simulink model "Motor_IMU_Test"  (R2026a)
settings: Solver=FixedStepAuto  StopTime=10  FixedStep=.001  EnableMultiTasking=on
InitFcn:
  | addpath('C:\Users\jpgre\OneDrive\Documents\ChatGPT\ETE 4851 Project\outputs\motor_imu');
libraries: stm32f4xxblockslib x4, stm32blockslib x3
settings Model: STM32="{\"DigitalPortWrite\":[{\"ID\":\"92\"},{\"ID\":\"93\"},{\"ID\":\"116\"}],\"PWMOutput\":{\"ID\":\"91\"},\"UARTWrite\":[{\"ID\":\"103\"},{\"ID\":\"110\"}],\"UARTRead\":{\"ID\":\"98\"}}"  SimulationMode=external  ExtModeTrigDuration=10  Creator=smboskovich  LastModifiedBy=jpgre
settings OptimizationCC: PassReuseOutputArgsThreshold=0.0  MaxStackSize=512
settings HardwareCC: ProdLargestAtomicInteger=Long  ProdLargestAtomicFloat=Double  ProdHWDeviceType=ARM Compatible->ARM Cortex-M
settings RTWCC: SystemTargetFile=ert.tlc  HardwareBoard=STM32F7xx Based (Double precision FPU)  TLCOptions=-aInlineSetEventsForThisBaseRateFcn=TLC_FALSE -aSuppressMultiTaskScheduler=TLC_FALSE -aRateBasedStepFcn=1  GenerateReport=on  Toolchain=GNU Tools for STM32  BuildConfiguration=Faster Runs  LaunchReport=on  Description=Embedded Coder
settings ERTTargetCC: ExtModeTransport=3.0  ExtModeStaticAllocSize=2048.0  DynamicArrayContainerType=coder::array  CodeReplacementLibrary=ARM Cortex-M  ERTCustomFileBanners=off  SupportContinuousTime=on  SupportNonInlinedSFcns=on  ModelStepFunctionPrototypeControlCompliant=off

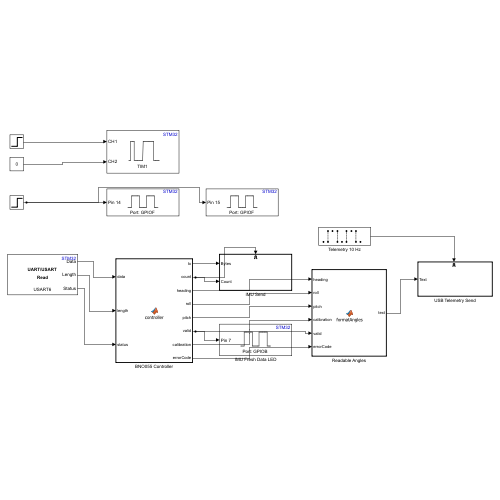
[thumbnail: Simulink's stored preview of the top-level diagram]
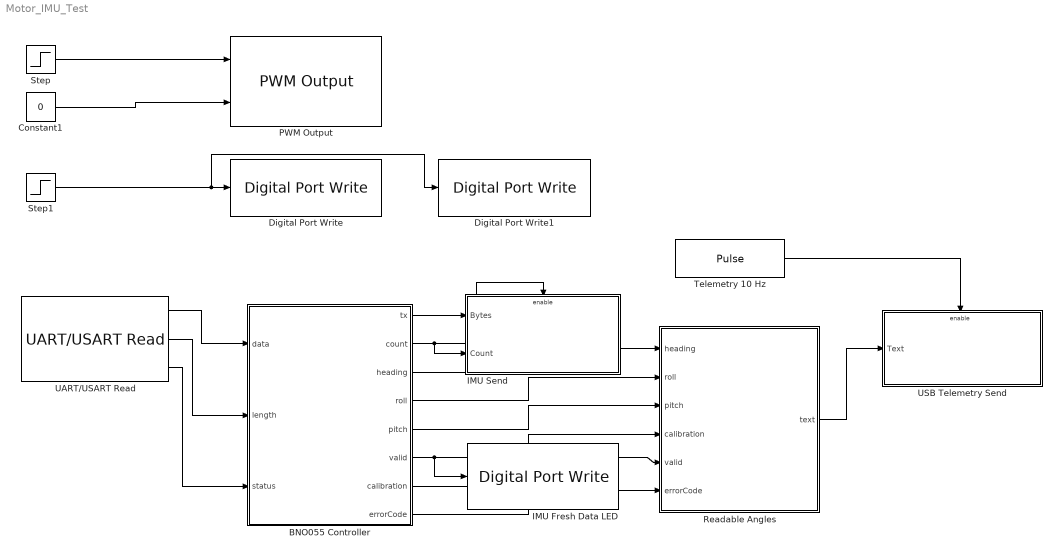
== system Motor_IMU_Test ==
  BNO055 Controller : MATLAB Function  TreatAsAtomicUnit=on
  Constant1 : Constant  Value=0
  Digital Port Write : stm32f4xxblockslib/Digital Port Write  PortName=GPIOF  PinNumber=[14]  ReadOperation=off  IOAsArray=off  EnableSimPort=off  hoistedMaskSrc=ECSoC/ECSimCodegen/Digital Port Write
      settings: LibrarySourceBlock=stm32h7xxblockslib/Digital Port Write
  Digital Port Write1 : stm32f4xxblockslib/Digital Port Write  PortName=GPIOF  PinNumber=[15]  ReadOperation=off  IOAsArray=off  EnableSimPort=off  hoistedMaskSrc=ECSoC/ECSimCodegen/Digital Port Write
      settings: LibrarySourceBlock=stm32h7xxblockslib/Digital Port Write
  IMU Fresh Data LED : stm32f4xxblockslib/Digital Port Write  PortName=GPIOB  PinNumber=7  ReadOperation=off  IOAsArray=off  EnableSimPort=off  hoistedMaskSrc=ECSoC/ECSimCodegen/Digital Port Write
      settings: LibrarySourceBlock=stm32h7xxblockslib/Digital Port Write
  IMU Send : Subsystem
  PWM Output : stm32f4xxblockslib/PWM Output  ProcessorFamily=STM32G4  TimerModule=TIM1  DutycycleUnits=Percentage  EnableChannel1=on  EnableCaptureCompare1Input=off  EnableCaptureCompare1ComplementaryInput=off  EnableOutputCompare1ModeInput=off  EnableChannel2=on  EnableCaptureCompare2Input=off  EnableCaptureCompare2ComplementaryInput=off  EnableOutputCompare2ModeInput=off  EnableChannel3=off  EnableCaptureCompare3Input=off  EnableCaptureCompare3ComplementaryInput=off  EnableOutputCompare3ModeInput=off  EnableChannel4=off  EnableCaptureCompare4Input=off  EnableCaptureCompare4ComplementaryInput=off  EnableOutputCompare4ModeInput=off  EnableChannel5=off  EnableCaptureCompare5Input=off  EnableOutputCompare5ModeInput=off  EnableChannel6=off  EnableCaptureCompare6Input=off  EnableOutputCompare6ModeInput=off  EnableCounterInput=off  EnableMainOutputInput=off  EnableFrequencyInput=off  SetRCAfterCE=off  OutputDirection=off  OutputMainOutputEnableStatus=off  SampleTime=0.1  EnableSimPort=off  EnableUpdateEvent=off  EnableCaptureCompare1Event=off  EnableCaptureCompare2Event=off  EnableCaptureCompare3Event=off  EnableCaptureCompare4Event=off  EnableTriggerEvent=off  EnableBreakEvent=off  EnableBreakEvent2=off  hoistedMaskSrc=ECSoC/ECSimCodegen/PWM Output
      settings: LibrarySourceBlock=stm32h7xxblockslib/PWM Output
  Readable Angles : MATLAB Function  TreatAsAtomicUnit=on
  Step : Step  Time=2  FinalValue=50  SampleTime=0.01
  Step1 : Step  Time=3  InitialValue=1  SampleTime=0.01
  Telemetry 10 Hz : DiscretePulseGenerator  Period=100  SampleTime=0.001
  UART/USART Read : stm32blockslib/UART//USART Read  UARTModule=USART6  DataType=uint8  DataLength=1  BlockingMode=off  BlockingTimeout=0.1  OutputLength=on  OutputStatus=on  SampleTime=0.001
  USB Telemetry Send : Subsystem
  wires:
  UART/USART Read/1 -> BNO055 Controller/1(data)
  UART/USART Read/2 -> BNO055 Controller/2(length)
  UART/USART Read/3 -> BNO055 Controller/3(status)
  BNO055 Controller/1(tx) -> IMU Send/1(Bytes)
  BNO055 Controller/2(count) -> IMU Send/2(Count), IMU Send/Enable
  BNO055 Controller/3(heading) -> Readable Angles/1(heading)
  BNO055 Controller/4(roll) -> Readable Angles/2(roll)
  BNO055 Controller/5(pitch) -> Readable Angles/3(pitch)
  BNO055 Controller/7(calibration) -> Readable Angles/4(calibration)
  BNO055 Controller/6(valid) -> Readable Angles/5(valid), IMU Fresh Data LED/1
  BNO055 Controller/8(errorCode) -> Readable Angles/6(errorCode)
  Readable Angles/1(text) -> USB Telemetry Send/1(Text)
  Telemetry 10 Hz/1 -> USB Telemetry Send/Enable
  Step/1 -> PWM Output/1
  Constant1/1 -> PWM Output/2
  Step1/1 -> Digital Port Write/1, Digital Port Write1/1

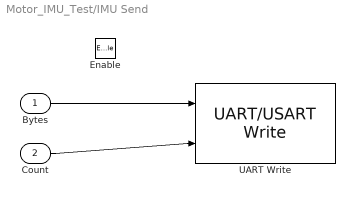
== system Motor_IMU_Test/IMU Send ==
  Bytes : Inport
  Count : Inport  Port=2
  Enable : EnablePort
  UART Write : stm32blockslib/UART//USART Write  UARTModule=USART6  LengthOfDataToSend=on  BlockingMode=off  BlockingTimeout=0.1  OutputStatus=off
  wires:
  Bytes/1 -> UART Write/1
  Count/1 -> UART Write/2

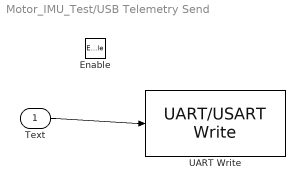
== system Motor_IMU_Test/USB Telemetry Send ==
  Text : Inport
  Enable : EnablePort
  UART Write : stm32blockslib/UART//USART Write  UARTModule=USART3  LengthOfDataToSend=off  BlockingMode=off  BlockingTimeout=0.1  OutputStatus=off
  wires:
  Text/1 -> UART Write/1

== matlab function Motor_IMU_Test/Readable Angles ==
  data: heading input; text output; roll input; pitch input; calibration input; valid input; errorCode input
function text = formatAngles(heading,roll,pitch,calibration,valid,errorCode)
text = bno055_text(heading,roll,pitch,calibration,valid,errorCode);
end

== matlab function Motor_IMU_Test/BNO055 Controller ==
  data: data input; tx output; length input; status input; count output; heading output; roll output; pitch output; valid output; calibration output; errorCode output
function [tx,count,heading,roll,pitch,valid,calibration,errorCode] = controller(data,length,status)
[tx,count,heading,roll,pitch,valid,calibration,errorCode] = bno055_controller(data,length,status);
end
